simulink model "PROJECT_32QAMSIMULINK"  (R2024a)
settings: Solver=VariableStepAuto  StartTime=0.0  StopTime=10.0  RelTol=1e-3
undefined symbols (not defined in the file or in its folder): doppler
libraries: commchan3 x2, commdigbbndam3 x2, commsink2 x1, commrandsrc3 x1
settings Model: Creator=JK JENA  LastModifiedBy=JK JENA

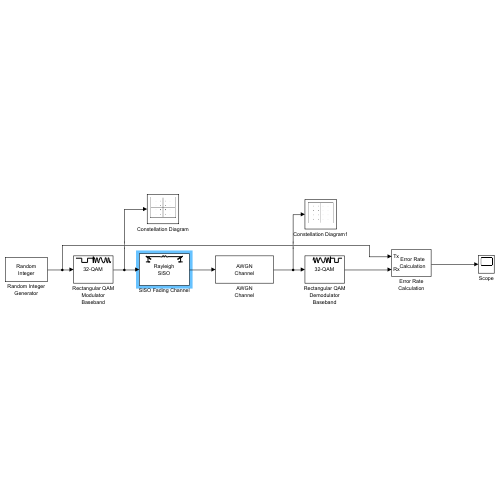
[thumbnail: Simulink's stored preview of the top-level diagram]
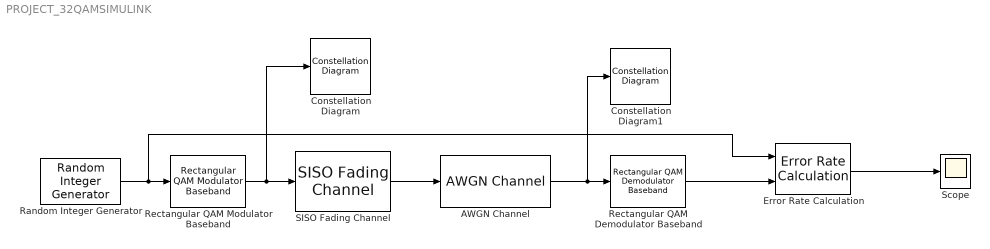
== system PROJECT_32QAMSIMULINK ==
  AWGN Channel : commchan3/AWGN Channel  LegacyMode=off  NoiseMethod="Signal to noise ratio  (Eb/No)"  noiseMode="Signal to noise ratio  (SNR)"  EbNo=12  EsNo=10  SNR=10  BitsPerSymbol=5  SignalPower=1  SamplesPerSymbol=1  SymbolPeriod=1  VarianceSource=Parameter  Variance=1  RandomStream=Global stream  Seed=67  SimulateUsing=Interpreted execution
  Constellation Diagram : ConstellationDiagram  WindowPosition=[817.000000,109.000000,600.000000,600.000000,]  Visible=on  ScopeFrameLocation=window
  Constellation Diagram1 : ConstellationDiagram  WindowPosition=[193.000000,109.000000,600.000000,600.000000,]  Visible=on  ScopeFrameLocation=window
  Error Rate Calculation : commsink2/Error Rate Calculation  N=0  st_delay=0  cp_mode=Entire frame  subframe=[]  PMode=Port  WsName=ErrorVec  RsMode2=off  stop=on  numErr=1000  maxBits=1e7
  Random Integer Generator : commrandsrc3/Random Integer Generator  SetSize=32  SeedSource=Auto  Seed=0  SampleTime=1  SamplesPerFrame=1000  OutputDataType=uint32  SimulateUsing=Interpreted execution
  Rectangular QAM Demodulator Baseband : commdigbbndam3/Rectangular QAM Demodulator Baseband  M=32  OutType=Integer  DecType=Hard decision  VarSource=Dialog  Variance=1  Dec=Gray  Mapping=[0:15]  PowType=Average Power  MinDist=2  AvgPow=1  PeakPow=1  Ph=0  outDtype1=Inherit via internal rule  outDtype2=Inherit via internal rule  derotateFactorWordLen=16  derotateFactorDataTypeStr=Inherit: Same word length as input  derotateFactorLastDataTypeStr=Inherit: Same word length as input  denormFactorWordLen=16  denormFactorDataTypeStr=Inherit: Same word length as input  denormFactorLastDataTypeStr=Inherit: Same word length as input  prodOutWordLen=32  prodOutOverflowMode=Saturate  prodOutRoundingMode=Floor  prodOutOvFlMode=on  prodOutOvFlModeLastStrValue=on  sumWordLen=32
  Rectangular QAM Modulator Baseband : commdigbbndam3/Rectangular QAM Modulator Baseband  M=32  InType=Integer  Enc=Gray  Mapping=[0:15]  PowType=Average Power  MinDist=2  AvgPow=1  PeakPow=1  Ph=0  outDtype=Inherit via back propagation  outWordLen=16  outUDDataType=sfix(16)  outFracLenMode=Best precision  outFracLen=15  outDataTypeStr=Inherit: Inherit via back propagation  outLastDataTypeStr=Inherit: Inherit via back propagation
  SISO Fading Channel : commchan3/SISO Fading Channel  InheritSampleRate=on  SampleRate=1  PathDelays=0  AveragePathGains=0  NormalizePathGains=on  FadingDistribution=Rayleigh  KFactor=3  DirectPathDopplerShift=0  DirectPathInitialPhase=0  MaximumDopplerShift=0  DopplerSpectrum=doppler('Jakes')  RandomStream=mt19937ar with seed  Seed=92  PathGainsOutputPort=off  ChannelFilterDelayOutputPort=off  SimulateUsing=Interpreted execution  Visualization=Off  PathsForDopplerDisplay=1  SamplesToDisplay=25%
  Scope : Scope
  wires:
  Rectangular QAM Modulator Baseband/1 -> Constellation Diagram/1, SISO Fading Channel/1
  SISO Fading Channel/1 -> AWGN Channel/1
  AWGN Channel/1 -> Constellation Diagram1/1, Rectangular QAM Demodulator Baseband/1
  Rectangular QAM Demodulator Baseband/1 -> Error Rate Calculation/2
  Random Integer Generator/1 -> Error Rate Calculation/1, Rectangular QAM Modulator Baseband/1
  Error Rate Calculation/1 -> Scope/1
